simulink subsystem "format_can_id"  (R2025a)
settings: Solver=VariableStepAuto  StartTime=0.0  StopTime=10.0  RelTol=1e-3
settings Model: Creator=upattacini  LastModifiedBy=mfussi
settings DebuggingCC: UnconnectedInputMsg=warning  UnconnectedOutputMsg=warning  UnconnectedLineMsg=warning
settings ModelReferenceCC: EnableRefExpFcnMdlSchedulingChecks=on
settings RTWCC: GPUComputeCapability=3.5  DLArmComputeVersion=19.05

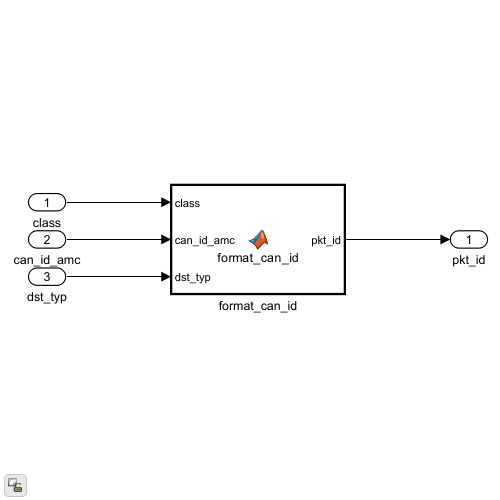
[thumbnail: Simulink's stored preview of the top-level diagram]
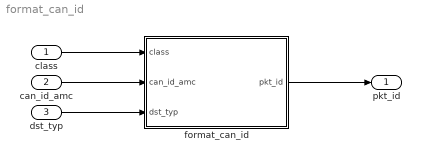
== system format_can_id ==
  class : Inport
  can_id_amc : Inport  Port=2
  dst_typ : Inport  Port=3
  format_can_id : MATLAB Function  TreatAsAtomicUnit=on
  pkt_id : Outport
  wires:
  dst_typ/1 -> format_can_id/3(dst_typ)
  format_can_id/1(pkt_id) -> pkt_id/1
  can_id_amc/1 -> format_can_id/2(can_id_amc)
  class/1 -> format_can_id/1(class)

== matlab function format_can_id/format_can_id ==
  data: class input uint8; pkt_id output uint16; can_id_amc input uint8; dst_typ input uint8
function pkt_id = format_can_id(class, can_id_amc, dst_typ)

class_int = uint16(class);
can_id_amc_int = uint16(can_id_amc);
dst_typ_int = uint16(dst_typ);
pkt_id = uint16(0);
pkt_id = bitor(pkt_id, bitshift(class_int, 8));
pkt_id = bitor(bitshift(can_id_amc_int,4), pkt_id);
pkt_id = bitor(dst_typ_int, pkt_id);
